simulink model "ASM_Traffic_A11"  (R2026a)
settings: Solver=ode1  StartTime=SIM.tstart.v  StopTime=SIM.tend.v  FixedStep=SIM.StepSize.v
PostLoadFcn:
  | if any(exist('dsrtsu_mdlpostloadfcn', 'file') ~= 0), dsrtsu_mdlpostloadfcn('Execute', bdroot); end
  | try, asm_mdl_postloadfcn(bdroot, 'UpdateModel', 3600); catch, disp(lasterr); end,
InitFcn:
  | , if any(exist('rtifpga_mdlclblib', 'file') ~= 0), rtifpga_mdlclblib('Init', bdroot); end,
  | , if any(exist('dsmpb_private', 'file') ~= 0), dsmpb_private('dsmpb_mdlclblib', 'Init', bdroot); end,
undefined symbols (not defined in the file): _to_, a0b2, ASM_BrakeHydraulics_DemoSystems, ASM_VehicleDynamics_DemoSystems, b98103fe8ad365046cd0, BrakeCircuit, controllerConfig, CPT, Crankshaft, DiscIntNeverNeededParam, dsmsi, FinalDriveAssembly, instance, MDL, ModeSignals, mu, Pos_BrakePedal_Maneuver, rad, RefSignals, s_to_rpm, SIM, SoftECU, Suspension, Tire, Transmission
libraries: ASM_Traffic_lib x135, simulink x98, ASM_Utils_lib x77, ASM_VehicleDynamics_lib x70, ASM_Environment_lib x22, dsmpblib x20, dsmsilib x15, MDLD_Utils_lib x10, ASM_BrakeHydraulics_lib x3, sl_discontinuities x2
(part 34 of 63)

== system ASM_Traffic_A11/DomainControl/DriverAssistance/Interface_In/ModelSignals/m_TotalVehicle[kg]_ ==
  In1 : Inport
  Gain : Gain  SaturateOnIntegerOverflow=on  OutDataTypeStr=Inherit: Same as input  ParamDataTypeStr=Inherit: Same as input
  Out1 : Outport  VectorParamsAs1DForOutWhenUnconnected=off
  wires:
  In1/1 -> Gain/1
  Gain/1 -> Out1/1

== system ASM_Traffic_A11/DomainControl/DriverAssistance/Interface_In/ModelSignals/r_Dyn_Tire[FL;FR;RL;RR][m]_ ==
  In1 : Inport
  Gain : Gain  SaturateOnIntegerOverflow=on  OutDataTypeStr=Inherit: Same as input  ParamDataTypeStr=Inherit: Same as input
  Out1 : Outport  VectorParamsAs1DForOutWhenUnconnected=off
  wires:
  In1/1 -> Gain/1
  Gain/1 -> Out1/1

== system ASM_Traffic_A11/DomainControl/DriverAssistance/Interface_In/ModelSignals/s_Fellows_Ref[m]_ ==
  In1 : Inport
  Gain : Gain  SaturateOnIntegerOverflow=on  OutDataTypeStr=Inherit: Same as input  ParamDataTypeStr=Inherit: Same as input
  Out1 : Outport  VectorParamsAs1DForOutWhenUnconnected=off
  wires:
  In1/1 -> Gain/1
  Gain/1 -> Out1/1

== system ASM_Traffic_A11/DomainControl/DriverAssistance/Interface_In/ModelSignals/s_Vehicle_Road[m]_ ==
  In1 : Inport
  Gain : Gain  SaturateOnIntegerOverflow=on  OutDataTypeStr=Inherit: Same as input  ParamDataTypeStr=Inherit: Same as input
  Out1 : Outport  VectorParamsAs1DForOutWhenUnconnected=off
  wires:
  In1/1 -> Gain/1
  Gain/1 -> Out1/1

== system ASM_Traffic_A11/DomainControl/DriverAssistance/Interface_In/ModelSignals/v_Rel_Fellows[m|s]_ ==
  In1 : Inport
  Gain : Gain  SaturateOnIntegerOverflow=on  OutDataTypeStr=Inherit: Same as input  ParamDataTypeStr=Inherit: Same as input
  Out1 : Outport  VectorParamsAs1DForOutWhenUnconnected=off
  wires:
  In1/1 -> Gain/1
  Gain/1 -> Out1/1

== system ASM_Traffic_A11/DomainControl/DriverAssistance/Interface_In/ModelSignals/v_Vehicle[km|h]_ ==
  In1 : Inport
  Gain : Gain  SaturateOnIntegerOverflow=on  OutDataTypeStr=Inherit: Same as input  ParamDataTypeStr=Inherit: Same as input
  Out1 : Outport  VectorParamsAs1DForOutWhenUnconnected=off
  wires:
  In1/1 -> Gain/1
  Gain/1 -> Out1/1

== system ASM_Traffic_A11/DomainControl/DriverAssistance/Interface_In/ModelSignals/v_x_Vehicle_CoG[km|h]_ ==
  In1 : Inport
  Gain : Gain  SaturateOnIntegerOverflow=on  OutDataTypeStr=Inherit: Same as input  ParamDataTypeStr=Inherit: Same as input
  Out1 : Outport  VectorParamsAs1DForOutWhenUnconnected=off
  wires:
  In1/1 -> Gain/1
  Gain/1 -> Out1/1

== system ASM_Traffic_A11/DomainControl/DriverAssistance/Interface_Out/Animation/Dist_Long[m]_ ==
  In1 : Inport
  Gain : Gain  SaturateOnIntegerOverflow=on  OutDataTypeStr=Inherit: Same as input  ParamDataTypeStr=Inherit: Same as input
  Out1 : Outport  VectorParamsAs1DForOutWhenUnconnected=off
  wires:
  In1/1 -> Gain/1
  Gain/1 -> Out1/1

== system ASM_Traffic_A11/DomainControl/DriverAssistance/Interface_Out/Animation/Distance_Set[m]_ ==
  In1 : Inport
  Gain : Gain  SaturateOnIntegerOverflow=on  OutDataTypeStr=Inherit: Same as input  ParamDataTypeStr=Inherit: Same as input
  Out1 : Outport  VectorParamsAs1DForOutWhenUnconnected=off
  wires:
  In1/1 -> Gain/1
  Gain/1 -> Out1/1

== system ASM_Traffic_A11/DomainControl/DriverAssistance/Interface_Out/Animation/State_ACC[0Off|1On]_ ==
  In1 : Inport
  Gain : Gain  SaturateOnIntegerOverflow=on  OutDataTypeStr=Inherit: Same as input  ParamDataTypeStr=Inherit: Same as input
  Out1 : Outport  VectorParamsAs1DForOutWhenUnconnected=off
  wires:
  In1/1 -> Gain/1
  Gain/1 -> Out1/1

== system ASM_Traffic_A11/DomainControl/DriverAssistance/Interface_Out/Animation/Target_Detected[0|1]_ ==
  In1 : Inport
  Gain : Gain  SaturateOnIntegerOverflow=on  OutDataTypeStr=Inherit: Same as input  ParamDataTypeStr=Inherit: Same as input
  Out1 : Outport  VectorParamsAs1DForOutWhenUnconnected=off
  wires:
  In1/1 -> Gain/1
  Gain/1 -> Out1/1

== system ASM_Traffic_A11/DomainControl/DriverAssistance/Interface_Out/Animation/v_Set[km|h]_ ==
  In1 : Inport
  Gain : Gain  SaturateOnIntegerOverflow=on  OutDataTypeStr=Inherit: Same as input  ParamDataTypeStr=Inherit: Same as input
  Out1 : Outport  VectorParamsAs1DForOutWhenUnconnected=off
  wires:
  In1/1 -> Gain/1
  Gain/1 -> Out1/1

== system ASM_Traffic_A11/DomainControl/DriverAssistance/Interface_Out/Control_ModelSignals/ACC_State[1OFF|2Standby|3ON]_ ==
  In1 : Inport
  Gain : Gain  SaturateOnIntegerOverflow=on  OutDataTypeStr=Inherit: Same as input  ParamDataTypeStr=Inherit: Same as input
  Out1 : Outport  VectorParamsAs1DForOutWhenUnconnected=off
  wires:
  Gain/1 -> Out1/1
  In1/1 -> Gain/1

== system ASM_Traffic_A11/DomainControl/DriverAssistance/Interface_Out/Control_ModelSignals/AEB[0|1]_ ==
  In1 : Inport
  Gain : Gain  SaturateOnIntegerOverflow=on  OutDataTypeStr=Inherit: Same as input  ParamDataTypeStr=Inherit: Same as input
  Out1 : Outport  VectorParamsAs1DForOutWhenUnconnected=off
  wires:
  In1/1 -> Gain/1
  Gain/1 -> Out1/1

== system ASM_Traffic_A11/DomainControl/DriverAssistance/Interface_Out/Control_ModelSignals/Driver_Override_ACC_Active[0Off|1On]_ ==
  In1 : Inport
  Gain : Gain  SaturateOnIntegerOverflow=on  OutDataTypeStr=Inherit: Same as input  ParamDataTypeStr=Inherit: Same as input
  Out1 : Outport  VectorParamsAs1DForOutWhenUnconnected=off
  wires:
  Gain/1 -> Out1/1
  In1/1 -> Gain/1

== system ASM_Traffic_A11/DomainControl/DriverAssistance/Interface_Out/Control_ModelSignals/Driver_Override_ACC_Reason[0NoOverride|1BrakePedal|2AccPedal]_ ==
  In1 : Inport
  Gain : Gain  SaturateOnIntegerOverflow=on  OutDataTypeStr=Inherit: Same as input  ParamDataTypeStr=Inherit: Same as input
  Out1 : Outport  VectorParamsAs1DForOutWhenUnconnected=off
  wires:
  Gain/1 -> Out1/1
  In1/1 -> Gain/1

== system ASM_Traffic_A11/DomainControl/DriverAssistance/Interface_Out/Control_ModelSignals/Enable_Trq_Decrease_ACC[0|1]_ ==
  In1 : Inport
  Gain : Gain  SaturateOnIntegerOverflow=on  OutDataTypeStr=Inherit: Same as input  ParamDataTypeStr=Inherit: Same as input
  Out1 : Outport  VectorParamsAs1DForOutWhenUnconnected=off
  wires:
  In1/1 -> Gain/1
  Gain/1 -> Out1/1

== system ASM_Traffic_A11/DomainControl/DriverAssistance/Interface_Out/Control_ModelSignals/Enable_Trq_Increase_ACC[0|1]_ ==
  In1 : Inport
  Gain : Gain  SaturateOnIntegerOverflow=on  OutDataTypeStr=Inherit: Same as input  ParamDataTypeStr=Inherit: Same as input
  Out1 : Outport  VectorParamsAs1DForOutWhenUnconnected=off
  wires:
  In1/1 -> Gain/1
  Gain/1 -> Out1/1

== system ASM_Traffic_A11/DomainControl/DriverAssistance/Interface_Out/Control_ModelSignals/FCW[0|1]_ ==
  In1 : Inport
  Gain : Gain  SaturateOnIntegerOverflow=on  OutDataTypeStr=Inherit: Same as input  ParamDataTypeStr=Inherit: Same as input
  Out1 : Outport  VectorParamsAs1DForOutWhenUnconnected=off
  wires:
  In1/1 -> Gain/1
  Gain/1 -> Out1/1

== system ASM_Traffic_A11/DomainControl/DriverAssistance/Interface_Out/Control_ModelSignals/Trq_DecreaseRequest_ACC[Nm]_ ==
  In1 : Inport
  Gain : Gain  SaturateOnIntegerOverflow=on  OutDataTypeStr=Inherit: Same as input  ParamDataTypeStr=Inherit: Same as input
  Out1 : Outport  VectorParamsAs1DForOutWhenUnconnected=off
  wires:
  In1/1 -> Gain/1
  Gain/1 -> Out1/1

== system ASM_Traffic_A11/DomainControl/DriverAssistance/Interface_Out/Control_ModelSignals/Trq_IncreaseRequest_ACC[Front;Rear][Nm]_ ==
  In1 : Inport
  Gain : Gain  SaturateOnIntegerOverflow=on  OutDataTypeStr=Inherit: Same as input  ParamDataTypeStr=Inherit: Same as input
  Out1 : Outport  VectorParamsAs1DForOutWhenUnconnected=off
  wires:
  In1/1 -> Gain/1
  Gain/1 -> Out1/1

== system ASM_Traffic_A11/DomainControl/DriverAssistance/Interface_Out/Control_ModelSignals/Trq_IncreaseRequest_ACC[Nm]_ ==
  In1 : Inport
  Gain : Gain  SaturateOnIntegerOverflow=on  OutDataTypeStr=Inherit: Same as input  ParamDataTypeStr=Inherit: Same as input
  Out1 : Outport  VectorParamsAs1DForOutWhenUnconnected=off
  wires:
  In1/1 -> Gain/1
  Gain/1 -> Out1/1

== system ASM_Traffic_A11/DomainControl/DriverAssistance/SignalInterface/ASMSignalInterface/signal_structure ==
  ASMSignalBus : Inport
  BusSelector_1 : BusSelector  OutputSignals=Controller_ACC,Interface_ACC,Operator_Interface_ACC,Target_Selection_ACC
  ContentID : Constant  Value=814723687
  Controller_ACC : BusSelector  OutputSignals=State_ACC[0Off|1On],Sw_ACC_Distance[s],Control_Mode_ACC[0Off|1CC|2DC],v_Set_CC[km|h],v_Set_DC[km|h],v_Set[km|h],a_x_Set[m|s2],a_x_UpperLimit[m|s2],a_x_LowerLimit[m|s2],a_x_RisingRateMax[m|s3],a_x_FallingRateMax[m|s3]s,Distance_Set[m],Dist_Ref_Vehicle[m],FCW[0Off|1On],AEB[0Off|1On],TTC[s],Collision[0Off|1On],Sw_BrakeMode[1Comfort|2AEBOnly|3AEBOff],Enable_Trq_Brake_ACC[0|1],Enable_Trq_Engine_ACC[0|1]
  DataTypeConversion_17 : DataTypeConversion  OutDataTypeStr=double
  InfoBlock : Subsystem
      mask Display: fprintf('Structural changes of the signal bus require an update \nof the ''ASMSignalCollector'' block. \n\nTo start the update process double click the parent block.\n\n WARNING:\n During update this subsystem will be cleared completely')
  Interface_ACC : BusSelector  OutputSignals=Trq_Request_Engine_ACC[Nm],Trq_Request_Engine_ACC[Front;Rear][Nm],Trq_Request_Brake_ACC[Nm]
  MDLD_DATA_CAPTURE : MDLD_Utils_lib/ModelDeskPlotInterface/DataCapture_Sfcn/MDLD_DATA_CAPTURE  inputPortWidth=70  measurementSignals=[0 0 0 0 0 0 0 0 0 0 0 0 0 0 0 0 0 0 0 0 0 0 0 0 0 0 0 0 0 0 0 0 0 0 0 0 0 0 0 0 0 0 0 0 0 0 0 0 0 0 0 0 0 0 0 0 0 0 0 0 0 0 0 0 0 0 0 0 0 0]  downsampling=1  samplingPeriod=SIM.StepSize.v  uuid=0  ASMProperties=struct('Name','mdld_data_capture','Version','1.0','Library','mdld_utils_lib')  startTriggerDelay=0  startTriggerLogic=0  startTriggerCount=0  startTriggerConditions=[0,0,0,0,0,0,0,0,0]  stopTriggerDelay=0  stopTriggerLogic=0  stopTriggerCount=0  stopTriggerConditions=[0,0,0,0,0,0,0,0,0]  ContentID_RefStruct=814723687
  Operator_Interface_ACC : BusSelector  OutputSignals=Sw_ACC_On[0Off|1On],Sw_ACC_Off[0Off|1On],Sw_ACC_Cancel[0Off|1On],Sw_ACC_Resume[0Off|1On],Sw_ACC_Speed_Set[0Off|1On],Sw_ACC_Speed_Increase[0Off|1On],Sw_ACC_Speed_Decrease[0Off|1On],ACC_State[1OFF|2Standby|3ON],Driver_Override_ACC_Active[0Off|1On],Driver_Override_ACC_Reason[0NoOverride|1BrakePedal|2AccPedal],V_Set_CruiseControl[km|h]
  Reshape_22 : Reshape
  Reshape_38 : Reshape
  Reshape_39 : Reshape
  SignalFilter : Mux  Inputs=41
  SignalFilterGain : Gain
  Target_Selection_ACC : BusSelector  OutputSignals=Target_Detected[0|1],Dist_Long[m],v_Rel[m|s],InLaneCheck[0|1],LaneCrossingCheck[0|1],v_Rel_Road[m|s],s_Fellows_Near[m]
  Terminator : Terminator
  wires:
  ASMSignalBus/1 -> BusSelector_1/1
  BusSelector_1/1 -> Controller_ACC/1  "<Controller_ACC>"
  BusSelector_1/2 -> Interface_ACC/1  "<Interface_ACC>"
  BusSelector_1/3 -> Operator_Interface_ACC/1  "<Operator_Interface_ACC>"
  BusSelector_1/4 -> Target_Selection_ACC/1  "<Target_Selection_ACC>"
  ContentID/1 -> Terminator/1
  Controller_ACC/1 -> SignalFilter/1  "<State_ACC[0Off|1On]>"
  Controller_ACC/2 -> SignalFilter/2  "<Sw_ACC_Distance[s]>"
  Controller_ACC/3 -> SignalFilter/3  "<Control_Mode_ACC[0Off|1CC|2DC]>"
  Controller_ACC/4 -> SignalFilter/4  "<v_Set_CC[km|h]>"
  Controller_ACC/5 -> SignalFilter/5  "<v_Set_DC[km|h]>"
  Controller_ACC/6 -> SignalFilter/6  "<v_Set[km|h]>"
  Controller_ACC/7 -> SignalFilter/7  "<a_x_Set[m|s2]>"
  Controller_ACC/8 -> SignalFilter/8  "<a_x_UpperLimit[m|s2]>"
  Controller_ACC/9 -> SignalFilter/9  "<a_x_LowerLimit[m|s2]>"
  Controller_ACC/10 -> SignalFilter/10  "<a_x_RisingRateMax[m|s3]>"
  Controller_ACC/11 -> SignalFilter/11  "<a_x_FallingRateMax[m|s3]s>"
  Controller_ACC/12 -> SignalFilter/12  "<Distance_Set[m]>"
  Controller_ACC/13 -> SignalFilter/13  "<Dist_Ref_Vehicle[m]>"
  Controller_ACC/14 -> SignalFilter/14  "<FCW[0Off|1On]>"
  Controller_ACC/15 -> SignalFilter/15  "<AEB[0Off|1On]>"
  Controller_ACC/16 -> SignalFilter/16  "<TTC[s]>"
  Controller_ACC/17 -> DataTypeConversion_17/1  "<Collision[0Off|1On]>"
  DataTypeConversion_17/1 -> SignalFilter/17
  Controller_ACC/18 -> SignalFilter/18  "<Sw_BrakeMode[1Comfort|2AEBOnly|3AEBOff]>"
  Controller_ACC/19 -> SignalFilter/19  "<Enable_Trq_Brake_ACC[0|1]>"
  Controller_ACC/20 -> SignalFilter/20  "<Enable_Trq_Engine_ACC[0|1]>"
  Interface_ACC/1 -> SignalFilter/21  "<Trq_Request_Engine_ACC[Nm]>"
  Interface_ACC/2 -> Reshape_22/1  "<Trq_Request_Engine_ACC[Front;Rear][Nm]>"
  Reshape_22/1 -> SignalFilter/22
  Interface_ACC/3 -> SignalFilter/23  "<Trq_Request_Brake_ACC[Nm]>"
  Operator_Interface_ACC/1 -> SignalFilter/24  "<Sw_ACC_On[0Off|1On]>"
  Operator_Interface_ACC/2 -> SignalFilter/25  "<Sw_ACC_Off[0Off|1On]>"
  Operator_Interface_ACC/3 -> SignalFilter/26  "<Sw_ACC_Cancel[0Off|1On]>"
  Operator_Interface_ACC/4 -> SignalFilter/27  "<Sw_ACC_Resume[0Off|1On]>"
  Operator_Interface_ACC/5 -> SignalFilter/28  "<Sw_ACC_Speed_Set[0Off|1On]>"
  Operator_Interface_ACC/6 -> SignalFilter/29  "<Sw_ACC_Speed_Increase[0Off|1On]>"
  Operator_Interface_ACC/7 -> SignalFilter/30  "<Sw_ACC_Speed_Decrease[0Off|1On]>"
  Operator_Interface_ACC/8 -> SignalFilter/31  "<ACC_State[1OFF|2Standby|3ON]>"
  Operator_Interface_ACC/9 -> SignalFilter/32  "<Driver_Override_ACC_Active[0Off|1On]>"
  Operator_Interface_ACC/10 -> SignalFilter/33  "<Driver_Override_ACC_Reason[0NoOverride|1BrakePedal|2AccPedal]>"
  Operator_Interface_ACC/11 -> SignalFilter/34  "<V_Set_CruiseControl[km|h]>"
  Target_Selection_ACC/1 -> SignalFilter/35  "<Target_Detected[0|1]>"
  Target_Selection_ACC/2 -> SignalFilter/36  "<Dist_Long[m]>"
  Target_Selection_ACC/3 -> SignalFilter/37  "<v_Rel[m|s]>"
  Target_Selection_ACC/4 -> Reshape_38/1  "<InLaneCheck[0|1]>"
  Reshape_38/1 -> SignalFilter/38
  Target_Selection_ACC/5 -> Reshape_39/1  "<LaneCrossingCheck[0|1]>"
  Reshape_39/1 -> SignalFilter/39
  Target_Selection_ACC/6 -> SignalFilter/40  "<v_Rel_Road[m|s]>"
  Target_Selection_ACC/7 -> SignalFilter/41  "<s_Fellows_Near[m]>"
  SignalFilter/1 -> SignalFilterGain/1
  SignalFilterGain/1 -> MDLD_DATA_CAPTURE/1

== system ASM_Traffic_A11/DomainControl/DriverAssistance/SignalInterface/ExternalOutports/Select_Outport_Signals ==
  ASMSignalBus : Inport
  Bus Selector : BusSelector  OutputSignals=Controller_ACC,Interface_ACC,Operator_Interface_ACC,Target_Selection_ACC
  Controller_ACC : Outport  VectorParamsAs1DForOutWhenUnconnected=off
  Interface_ACC : Outport  Port=2  VectorParamsAs1DForOutWhenUnconnected=off
  Operator_Interface_ACC : Outport  Port=3  VectorParamsAs1DForOutWhenUnconnected=off
  Target_Selection_ACC : Outport  Port=4  VectorParamsAs1DForOutWhenUnconnected=off
  wires:
  ASMSignalBus/1 -> Bus Selector/1
  Bus Selector/1 -> Controller_ACC/1  "<Controller_ACC>"
  Bus Selector/2 -> Interface_ACC/1  "<Interface_ACC>"
  Bus Selector/3 -> Operator_Interface_ACC/1  "<Operator_Interface_ACC>"
  Bus Selector/4 -> Target_Selection_ACC/1  "<Target_Selection_ACC>"

== system ASM_Traffic_A11/DomainControl/StartSystem/Control/SoftECU_StartSystem/ASMSignalCollector ==
  Bus Creator1 : BusCreator  Inputs=1
  ASMSIgnalBus : Outport  VectorParamsAs1DForOutWhenUnconnected=off
  wires:
  [ASMBUS_START_BUTTON] -> Bus Creator1/1
  Bus Creator1/1 -> ASMSIgnalBus/1  "Control"

== system ASM_Traffic_A11/DomainControl/StartSystem/Control/SoftECU_StartSystem/DisableReset ==
  note: Start button is not reset, if crankshaft reset is disabled
  Reset_VehicleStates[0|1] : Inport
  Sw_CrankShaft_Reset[0Disabled|1Enabled] : Inport  Port=2
  MultiPortSwitch : MultiPortSwitch  DataPortOrder=Zero-based contiguous  Inputs=2  zeroidx=on
  NO_Reset : Constant  Value=0
  Reset[0|1] : Outport  VectorParamsAs1DForOutWhenUnconnected=off
  wires:
  MultiPortSwitch/1 -> Reset[0|1]/1
  Sw_CrankShaft_Reset[0Disabled|1Enabled]/1 -> MultiPortSwitch/1
  NO_Reset/1 -> MultiPortSwitch/2
  Reset_VehicleStates[0|1]/1 -> MultiPortSwitch/3

== system ASM_Traffic_A11/DomainControl/StartSystem/Control/Sw_ECU_Signals/State_StartButton[-2|-1|0|1|2|3] ==
  SoftECU : Inport
  RealECU : Inport  Port=2
  Const_State_StartButton[-2|-1|0|1|2|3] : Constant  Value=0
  MultiPortSwitch : MultiPortSwitch
  Sw_State_StartButton[1SoftECU|2RealECU|3Const] : Constant  Value=CPT.MDL_SW.Sw_State_StartButton.v
  State_StartButton[-2|-1|0|1|2|3] : Outport  VectorParamsAs1DForOutWhenUnconnected=off
  wires:
  Sw_State_StartButton[1SoftECU|2RealECU|3Const]/1 -> MultiPortSwitch/1
  SoftECU/1 -> MultiPortSwitch/2
  RealECU/1 -> MultiPortSwitch/3
  Const_State_StartButton[-2|-1|0|1|2|3]/1 -> MultiPortSwitch/4
  MultiPortSwitch/1 -> State_StartButton[-2|-1|0|1|2|3]/1

== system ASM_Traffic_A11/DomainControl/StartSystem/Control/Sw_ECU_Signals/Sw_Ignition[0|1] ==
  SoftECU : Inport
  RealECU : Inport  Port=2
  Const_Sw_Ignition[0|1] : Constant  Value=0
  MultiPortSwitch : MultiPortSwitch
  Sw_Ignition[1SoftECU|2RealECU|3Const] : Constant  Value=CPT.MDL_SW.Sw_Ignition.v
  Sw_Ignition[0|1] : Outport  VectorParamsAs1DForOutWhenUnconnected=off
  wires:
  MultiPortSwitch/1 -> Sw_Ignition[0|1]/1
  Const_Sw_Ignition[0|1]/1 -> MultiPortSwitch/4
  RealECU/1 -> MultiPortSwitch/3
  SoftECU/1 -> MultiPortSwitch/2
  Sw_Ignition[1SoftECU|2RealECU|3Const]/1 -> MultiPortSwitch/1

== system ASM_Traffic_A11/DomainControl/StartSystem/Control/Sw_ECU_Signals/Sw_StarterReq[0|1] ==
  SoftECU : Inport
  RealECU : Inport  Port=2
  Const_Sw_StarterReq[0|1] : Constant  Value=0
  MultiPortSwitch : MultiPortSwitch
  Sw_StarterReq[1SoftECU|2RealECU|3Const] : Constant  Value=CPT.MDL_SW.Sw_StarterReq.v
  Sw_StarterReq[0|1] : Outport  VectorParamsAs1DForOutWhenUnconnected=off
  wires:
  Sw_StarterReq[1SoftECU|2RealECU|3Const]/1 -> MultiPortSwitch/1
  SoftECU/1 -> MultiPortSwitch/2
  RealECU/1 -> MultiPortSwitch/3
  Const_Sw_StarterReq[0|1]/1 -> MultiPortSwitch/4
  MultiPortSwitch/1 -> Sw_StarterReq[0|1]/1

== system ASM_Traffic_A11/DomainControl/StartSystem/Control/UserInterface/ASMSignalBus_Control ==
  In : Inport
  Terminator_1 : Terminator
  tag scope: ASMBUS_StartSystem_Control=global
  wires:
  In/1 -> [ASMBUS_StartSystem_Control]  "Control"
  [ASMBUS_StartSystem_Control] -> Terminator_1/1

== system ASM_Traffic_A11/DomainControl/StartSystem/Control/UserInterface/DISP_Control ==
  In : Inport
  Interface_In : Inport  Port=2
  Bus Selector1 : BusSelector  OutputSignals=ExternalModel.State_Engine[0|1|2|3|4],ExternalModel.Mode_StartButtonState[1Stim|2SoftECU]
  Bus Selector3 : BusSelector  OutputSignals=StartButton.Flag_NotPressed_Pedal[0|1],StartButton.Sw_Ignition[0|1],StartButton.Sw_StarterReq[0|1],StartButton.State_StartButton[-2|-1|0|1|2|3]
  Flag_NotPressed_Pedal[0|1] : Subsystem
      mask Display: disp('')
  START_BUTTON : Scope  NumInputPorts=4
      settings: TimeSpan=5  DataLoggingMaxPoints=20000  DataLoggingDecimation=10  DataLoggingSaveFormat=Array
  StartStateButtonLogic : Subsystem
  State_StartButton[-2NotAuthorized|-1PowerOff|0Acc|1PowerOn|2StarterOn|3EngRunning] : Subsystem
      mask Display: disp('')
  Sw_Ignition[0|1] : Subsystem
      mask Display: disp('')
  Sw_StarterReq[0|1] : Subsystem
      mask Display: disp('')
  wires:
  Bus Selector3/3 -> Sw_StarterReq[0|1]/1(In1)  "<Sw_StarterReq[0|1]>"
  Bus Selector1/1 -> StartStateButtonLogic/2(State_Engine[0|1|2|3|4])  "<State_Engine[0|1|2|3|4]>"
  Bus Selector1/2 -> StartStateButtonLogic/3(Mode_StartButtonState[1Stim|2SoftECU])  "<Mode_StartButtonState[1Stim|2SoftECU]>"
  Flag_NotPressed_Pedal[0|1]/1(Out1) -> START_BUTTON/1  "Flag_NotPressed_Pedal[0|1]"
  StartStateButtonLogic/1(Out1) -> State_StartButton[-2NotAuthorized|-1PowerOff|0Acc|1PowerOn|2StarterOn|3EngRunning]/1(In1)
  State_StartButton[-2NotAuthorized|-1PowerOff|0Acc|1PowerOn|2StarterOn|3EngRunning]/1(Out1) -> START_BUTTON/4  "State_StartButton[-2NotAuthorized|-1PowerOff|0Acc|1PowerOn|2StarterOn|3EngRunning]"
  Sw_Ignition[0|1]/1(Out1) -> START_BUTTON/2  "Sw_Ignition[0|1]"
  Bus Selector3/2 -> Sw_Ignition[0|1]/1(In1)  "<Sw_Ignition[0|1]>"
  Sw_StarterReq[0|1]/1(Out1) -> START_BUTTON/3  "Sw_StarterReq[0|1]"
  Bus Selector3/4 -> StartStateButtonLogic/1(State_StartButton[-2|-1|0|1|2|3])  "<State_StartButton[-2|-1|0|1|2|3]>"
  Bus Selector3/1 -> Flag_NotPressed_Pedal[0|1]/1(In1)  "<Flag_NotPressed_Pedal[0|1]>"
  In/1 -> Bus Selector3/1
  Interface_In/1 -> Bus Selector1/1

== system ASM_Traffic_A11/DomainControl/StartSystem/Control/UserInterface/PAR_Control ==
  Bus Creator2 : BusCreator  Inputs=1
  State_KeyFob[1NotAuthorized|2Authorized] : Constant  Value=2
  Out : Outport  VectorParamsAs1DForOutWhenUnconnected=off
  wires:
  Bus Creator2/1 -> Out/1  "PAR2Control"
  State_KeyFob[1NotAuthorized|2Authorized]/1 -> Bus Creator2/1  "State_KeyFob[1NotAuthorized|2Authorized]"

== system ASM_Traffic_A11/DomainControl/StartSystem/Interface_In/ExternalSignals/ExternalECU_StartSystem ==
  State_StartButton[-2|-1|0|1|2|3] : Inport
  Sw_Ignition[0|1] : Inport  Port=2
  Sw_StarterReq[0|1] : Inport  Port=3
  Bus Creator4 : BusCreator  Inputs=3
  Out : Outport  VectorParamsAs1DForOutWhenUnconnected=off
  wires:
  State_StartButton[-2|-1|0|1|2|3]/1 -> Bus Creator4/1  "State_StartButton[-2|-1|0|1|2|3]"
  Bus Creator4/1 -> Out/1  "ExternalECU"
  Sw_Ignition[0|1]/1 -> Bus Creator4/2  "Sw_Ignition[0|1]"
  Sw_StarterReq[0|1]/1 -> Bus Creator4/3  "Sw_StarterReq[0|1]"

== system ASM_Traffic_A11/DomainControl/StartSystem/Interface_In/ModelSignals/Mode_StartButtonState[1Stim|2SoftECU]_ ==
  In1 : Inport
  DummyGain : Gain  SaturateOnIntegerOverflow=on  OutDataTypeStr=Inherit: Same as input  ParamDataTypeStr=Inherit: Same as input
  Out1 : Outport  VectorParamsAs1DForOutWhenUnconnected=off
  wires:
  In1/1 -> DummyGain/1
  DummyGain/1 -> Out1/1

== system ASM_Traffic_A11/DomainControl/StartSystem/Interface_In/ModelSignals/Mode_Transmission[1Manual|2Automatic]_ ==
  In1 : Inport
  DummyGain : Gain  SaturateOnIntegerOverflow=on  OutDataTypeStr=Inherit: Same as input  ParamDataTypeStr=Inherit: Same as input
  Out1 : Outport  VectorParamsAs1DForOutWhenUnconnected=off
  wires:
  In1/1 -> DummyGain/1
  DummyGain/1 -> Out1/1

== system ASM_Traffic_A11/DomainControl/StartSystem/Interface_In/ModelSignals/Pos_BrakePedal[%]_ ==
  In1 : Inport
  DummyGain : Gain  SaturateOnIntegerOverflow=on  OutDataTypeStr=Inherit: Same as input  ParamDataTypeStr=Inherit: Same as input
  Out1 : Outport  VectorParamsAs1DForOutWhenUnconnected=off
  wires:
  In1/1 -> DummyGain/1
  DummyGain/1 -> Out1/1

== system ASM_Traffic_A11/DomainControl/StartSystem/Interface_In/ModelSignals/Pos_ClutchPedal[%]_ ==
  In1 : Inport
  DummyGain : Gain  SaturateOnIntegerOverflow=on  OutDataTypeStr=Inherit: Same as input  ParamDataTypeStr=Inherit: Same as input
  Out1 : Outport  VectorParamsAs1DForOutWhenUnconnected=off
  wires:
  In1/1 -> DummyGain/1
  DummyGain/1 -> Out1/1

== system ASM_Traffic_A11/DomainControl/StartSystem/Interface_In/ModelSignals/Reset_States[0|1]_ ==
  In1 : Inport
  DummyGain : Gain  SaturateOnIntegerOverflow=on  OutDataTypeStr=Inherit: Same as input  ParamDataTypeStr=Inherit: Same as input
  Out1 : Outport  VectorParamsAs1DForOutWhenUnconnected=off
  wires:
  In1/1 -> DummyGain/1
  DummyGain/1 -> Out1/1

== system ASM_Traffic_A11/DomainControl/StartSystem/Interface_In/ModelSignals/SelectorLever[-3T|-2P|-1R|0N|1D]_ ==
  In1 : Inport
  DummyGain : Gain  SaturateOnIntegerOverflow=on  OutDataTypeStr=Inherit: Same as input  ParamDataTypeStr=Inherit: Same as input
  Out1 : Outport  VectorParamsAs1DForOutWhenUnconnected=off
  wires:
  In1/1 -> DummyGain/1
  DummyGain/1 -> Out1/1

== system ASM_Traffic_A11/DomainControl/StartSystem/Interface_In/ModelSignals/State_Engine[0|1|2|3|4]_ ==
  In1 : Inport
  DummyGain : Gain  SaturateOnIntegerOverflow=on  OutDataTypeStr=Inherit: Same as input  ParamDataTypeStr=Inherit: Same as input
  Out1 : Outport  VectorParamsAs1DForOutWhenUnconnected=off
  wires:
  In1/1 -> DummyGain/1
  DummyGain/1 -> Out1/1

== system ASM_Traffic_A11/DomainControl/StartSystem/Interface_In/ModelSignals/State_StartButton[-1PowerOff|0Acc|1PowerOn|2StarterOn]_ ==
  In1 : Inport
  DummyGain : Gain  SaturateOnIntegerOverflow=on  OutDataTypeStr=Inherit: Same as input  ParamDataTypeStr=Inherit: Same as input
  Out1 : Outport  VectorParamsAs1DForOutWhenUnconnected=off
  wires:
  In1/1 -> DummyGain/1
  DummyGain/1 -> Out1/1

== system ASM_Traffic_A11/DomainControl/StartSystem/Interface_In/ModelSignals/Sw_CrankShaft_Reset[0Disabled|1Enabled]_ ==
  In1 : Inport
  DummyGain : Gain  SaturateOnIntegerOverflow=on  OutDataTypeStr=Inherit: Same as input  ParamDataTypeStr=Inherit: Same as input
  Out1 : Outport  VectorParamsAs1DForOutWhenUnconnected=off
  wires:
  DummyGain/1 -> Out1/1
  In1/1 -> DummyGain/1

== system ASM_Traffic_A11/DomainControl/StartSystem/Interface_In/ModelSignals/Sw_ModelDeskPlottingInterface[0Disabled|1Enabled]_ ==
  In1 : Inport
  Gain : Gain
  Out1 : Outport
  wires:
  Gain/1 -> Out1/1
  In1/1 -> Gain/1

== system ASM_Traffic_A11/DomainControl/StartSystem/Interface_In/ModelSignals/Sw_ModelPortBlocks[0Disabled|1Enabled]_ ==
  In1 : Inport
  Gain : Gain
  Out1 : Outport
  wires:
  Gain/1 -> Out1/1
  In1/1 -> Gain/1

== system ASM_Traffic_A11/DomainControl/StartSystem/Interface_In/ModelSignals/Sw_StartButton[0Off|1On]_ ==
  In1 : Inport
  DummyGain : Gain  SaturateOnIntegerOverflow=on  OutDataTypeStr=Inherit: Same as input  ParamDataTypeStr=Inherit: Same as input
  Out1 : Outport  VectorParamsAs1DForOutWhenUnconnected=off
  wires:
  In1/1 -> DummyGain/1
  DummyGain/1 -> Out1/1

== system ASM_Traffic_A11/DomainControl/StartSystem/Interface_Out/Control_ModelSignals/State_StartButton[-2|-1|0|1|2|3]_ ==
  In1 : Inport
  DummyGain : Gain  SaturateOnIntegerOverflow=on  OutDataTypeStr=Inherit: Same as input  ParamDataTypeStr=Inherit: Same as input
  Out1 : Outport  VectorParamsAs1DForOutWhenUnconnected=off
  wires:
  DummyGain/1 -> Out1/1
  In1/1 -> DummyGain/1

== system ASM_Traffic_A11/DomainControl/StartSystem/Interface_Out/Control_ModelSignals/Sw_Ignition[0|1]_ ==
  In1 : Inport
  DummyGain : Gain  SaturateOnIntegerOverflow=on  OutDataTypeStr=Inherit: Same as input  ParamDataTypeStr=Inherit: Same as input
  Out1 : Outport  VectorParamsAs1DForOutWhenUnconnected=off
  wires:
  DummyGain/1 -> Out1/1
  In1/1 -> DummyGain/1

== system ASM_Traffic_A11/DomainControl/StartSystem/Interface_Out/Control_ModelSignals/Sw_StarterReq[0|1]_ ==
  In1 : Inport
  DummyGain : Gain  SaturateOnIntegerOverflow=on  OutDataTypeStr=Inherit: Same as input  ParamDataTypeStr=Inherit: Same as input
  Out1 : Outport  VectorParamsAs1DForOutWhenUnconnected=off
  wires:
  In1/1 -> DummyGain/1
  DummyGain/1 -> Out1/1

== system ASM_Traffic_A11/DomainControl/StartSystem/SignalInterface/ASMSignalInterface/signal_structure ==
  ASMSignalBus : Inport
  BusSelector_1 : BusSelector  OutputSignals=StartButton
  ContentID : Constant  Value=905791938
  DataTypeConversion_1 : DataTypeConversion  OutDataTypeStr=double
  InfoBlock : Subsystem
      mask Display: fprintf('Structural changes of the signal bus require an update \nof the ''ASMSignalCollector'' block. \n\nTo start the update process double click the parent block.\n\n WARNING:\n During update this subsystem will be cleared completely')
  MDLD_DATA_CAPTURE : MDLD_Utils_lib/ModelDeskPlotInterface/DataCapture_Sfcn/MDLD_DATA_CAPTURE  inputPortWidth=6  measurementSignals=[0 0 0 0 0 0]  downsampling=1  samplingPeriod=SIM.StepSize.v  uuid=0  ASMProperties=struct('Name','mdld_data_capture','Version','1.0','Library','mdld_utils_lib')  startTriggerDelay=0  startTriggerLogic=0  startTriggerCount=0  startTriggerConditions=[0,0,0,0,0,0,0,0,0]  stopTriggerDelay=0  stopTriggerLogic=0  stopTriggerCount=0  stopTriggerConditions=[0,0,0,0,0,0,0,0,0]  ContentID_RefStruct=905791938
  SignalFilter : Mux  Inputs=6
  SignalFilterGain : Gain
  StartButton : BusSelector  OutputSignals=Flag_NotPressed_Pedal[0|1],Lock[0|1],Sw_Acc[0|1],Sw_Ignition[0|1],Sw_StarterReq[0|1],State_StartButton[-2|-1|0|1|2|3]
  Terminator : Terminator
  wires:
  ASMSignalBus/1 -> BusSelector_1/1
  BusSelector_1/1 -> StartButton/1  "<StartButton>"
  ContentID/1 -> Terminator/1
  StartButton/1 -> DataTypeConversion_1/1  "<Flag_NotPressed_Pedal[0|1]>"
  DataTypeConversion_1/1 -> SignalFilter/1
  StartButton/2 -> SignalFilter/2  "<Lock[0|1]>"
  StartButton/3 -> SignalFilter/3  "<Sw_Acc[0|1]>"
  StartButton/4 -> SignalFilter/4  "<Sw_Ignition[0|1]>"
  StartButton/5 -> SignalFilter/5  "<Sw_StarterReq[0|1]>"
  StartButton/6 -> SignalFilter/6  "<State_StartButton[-2|-1|0|1|2|3]>"
  SignalFilter/1 -> SignalFilterGain/1
  SignalFilterGain/1 -> MDLD_DATA_CAPTURE/1

== system ASM_Traffic_A11/DomainControl/StartSystem/SignalInterface/ExternalOutports/Select_Outport_Signals ==
  ASMSignalBus : Inport
  Bus Selector : BusSelector  OutputSignals=StartButton.Flag_NotPressed_Pedal[0|1],StartButton.Lock[0|1],StartButton.Sw_Acc[0|1],StartButton.Sw_Ignition[0|1],StartButton.Sw_StarterReq[0|1],StartButton.State_StartButton[-2|-1|0|1|2|3]
  Flag_NotPressed_Pedal[0|1] : Outport  VectorParamsAs1DForOutWhenUnconnected=off
  Lock[0|1] : Outport  Port=2  VectorParamsAs1DForOutWhenUnconnected=off
  Sw_Acc[0|1] : Outport  Port=3  VectorParamsAs1DForOutWhenUnconnected=off
  Sw_Ignition[0|1] : Outport  Port=4  VectorParamsAs1DForOutWhenUnconnected=off
  Sw_StarterReq[0|1] : Outport  Port=5  VectorParamsAs1DForOutWhenUnconnected=off
  State_StartButton[-2|-1|0|1|2|3] : Outport  Port=6  VectorParamsAs1DForOutWhenUnconnected=off
  wires:
  ASMSignalBus/1 -> Bus Selector/1
  Bus Selector/1 -> Flag_NotPressed_Pedal[0|1]/1  "<Flag_NotPressed_Pedal[0|1]>"
  Bus Selector/2 -> Lock[0|1]/1  "<Lock[0|1]>"
  Bus Selector/3 -> Sw_Acc[0|1]/1  "<Sw_Acc[0|1]>"
  Bus Selector/4 -> Sw_Ignition[0|1]/1  "<Sw_Ignition[0|1]>"
  Bus Selector/5 -> Sw_StarterReq[0|1]/1  "<Sw_StarterReq[0|1]>"
  Bus Selector/6 -> State_StartButton[-2|-1|0|1|2|3]/1  "<State_StartButton[-2|-1|0|1|2|3]>"

== system ASM_Traffic_A11/DomainControl/TorqueManager/Control/UserInterface/ASMSignalBus_Control ==
  In : Inport
  Terminator_1 : Terminator
  tag scope: ASMBUS_TorqueManager_Control=global
  wires:
  In/1 -> [ASMBUS_TorqueManager_Control]  "Control"
  [ASMBUS_TorqueManager_Control] -> Terminator_1/1

== system ASM_Traffic_A11/DomainControl/TorqueManager/Control/UserInterface/DISP_Control ==
  In : Inport
  Terminator : Terminator
  wires:
  In/1 -> Terminator/1

== system ASM_Traffic_A11/DomainControl/TorqueManager/Control/UserInterface/PAR_Control ==
  Constant : Constant  Value=0
  Out : Outport  VectorParamsAs1DForOutWhenUnconnected=off
  wires:
  Constant/1 -> Out/1

== system ASM_Traffic_A11/DomainControl/TorqueManager/Interface_In/ModelSignals/Pos_BrakePedal[%]_ ==
  In1 : Inport
  DummyGain : Gain  SaturateOnIntegerOverflow=on  OutDataTypeStr=Inherit: Same as input  ParamDataTypeStr=Inherit: Same as input
  Out1 : Outport  VectorParamsAs1DForOutWhenUnconnected=off
  wires:
  DummyGain/1 -> Out1/1
  In1/1 -> DummyGain/1

== system ASM_Traffic_A11/DomainControl/TorqueManager/Interface_In/ModelSignals/State_Engine[0|1|2|3|4]_ ==
  In1 : Inport
  Gain : Gain  SaturateOnIntegerOverflow=on  OutDataTypeStr=Inherit: Same as input  ParamDataTypeStr=Inherit: Same as input
  Out1 : Outport  VectorParamsAs1DForOutWhenUnconnected=off
  wires:
  In1/1 -> Gain/1
  Gain/1 -> Out1/1

== system ASM_Traffic_A11/DomainControl/TorqueManager/Interface_In/ModelSignals/Sw_Ignition[0|1]_ ==
  In1 : Inport
  DummyGain : Gain  SaturateOnIntegerOverflow=on  OutDataTypeStr=Inherit: Same as input  ParamDataTypeStr=Inherit: Same as input
  Out1 : Outport  VectorParamsAs1DForOutWhenUnconnected=off
  wires:
  In1/1 -> DummyGain/1
  DummyGain/1 -> Out1/1

== system ASM_Traffic_A11/DomainControl/TorqueManager/Interface_In/ModelSignals/Sw_ModelDeskPlottingInterface[0Disabled|1Enabled]_ ==
  In1 : Inport
  Gain : Gain
  Out1 : Outport
  wires:
  Gain/1 -> Out1/1
  In1/1 -> Gain/1

== system ASM_Traffic_A11/DomainControl/TorqueManager/Interface_In/ModelSignals/Sw_ModelPortBlocks[0Disabled|1Enabled]_ ==
  In1 : Inport
  Gain : Gain
  Out1 : Outport
  wires:
  Gain/1 -> Out1/1
  In1/1 -> Gain/1

== system ASM_Traffic_A11/DomainControl/TorqueManager/Interface_In/ModelSignals/Sw_StarterReq[0|1]_ ==
  In1 : Inport
  DummyGain : Gain  SaturateOnIntegerOverflow=on  OutDataTypeStr=Inherit: Same as input  ParamDataTypeStr=Inherit: Same as input
  Out1 : Outport  VectorParamsAs1DForOutWhenUnconnected=off
  wires:
  DummyGain/1 -> Out1/1
  In1/1 -> DummyGain/1

== system ASM_Traffic_A11/DomainControl/TorqueManager/Interface_In/ModelSignals/Sw_Starter[0Off|1On]_ ==
  In1 : Inport
  DummyGain : Gain  SaturateOnIntegerOverflow=on  OutDataTypeStr=Inherit: Same as input  ParamDataTypeStr=Inherit: Same as input
  Out1 : Outport  VectorParamsAs1DForOutWhenUnconnected=off
  wires:
  In1/1 -> DummyGain/1
  DummyGain/1 -> Out1/1

== system ASM_Traffic_A11/DomainControl/TorqueManager/Interface_Out/Control_ModelSignals/ Mode_BSG[-1|0|1|2|3|4|5]_ ==
  In1 : Inport
  Gain : Gain  SaturateOnIntegerOverflow=on  OutDataTypeStr=Inherit: Same as input  ParamDataTypeStr=Inherit: Same as input
  Out1 : Outport  VectorParamsAs1DForOutWhenUnconnected=off
  wires:
  Gain/1 -> Out1/1
  In1/1 -> Gain/1

== system ASM_Traffic_A11/DomainControl/TorqueManager/Interface_Out/Control_ModelSignals/HybridMode_ICE[0Off|1OnIdle|2OnPower|3err]_ ==
  In1 : Inport
  Gain : Gain  SaturateOnIntegerOverflow=on  OutDataTypeStr=Inherit: Same as input  ParamDataTypeStr=Inherit: Same as input
  Out1 : Outport  VectorParamsAs1DForOutWhenUnconnected=off
  wires:
  In1/1 -> Gain/1
  Gain/1 -> Out1/1

== system ASM_Traffic_A11/DomainControl/TorqueManager/Interface_Out/Control_ModelSignals/Ignition_ICE[0Off|1On]_ ==
  In1 : Inport
  Gain : Gain  SaturateOnIntegerOverflow=on  OutDataTypeStr=Inherit: Same as input  ParamDataTypeStr=Inherit: Same as input
  Out1 : Outport  VectorParamsAs1DForOutWhenUnconnected=off
  wires:
  In1/1 -> Gain/1
  Gain/1 -> Out1/1

== system ASM_Traffic_A11/DomainControl/TorqueManager/Interface_Out/Control_ModelSignals/Pos_BrakePedal_Desired[%]_ ==
  In1 : Inport
  Gain : Gain  SaturateOnIntegerOverflow=on  OutDataTypeStr=Inherit: Same as input  ParamDataTypeStr=Inherit: Same as input
  Out1 : Outport  VectorParamsAs1DForOutWhenUnconnected=off
  wires:
  In1/1 -> Gain/1
  Gain/1 -> Out1/1

== system ASM_Traffic_A11/DomainControl/TorqueManager/Interface_Out/Control_ModelSignals/StarterReq_ICE[0Off|1On]_ ==
  In1 : Inport
  Gain : Gain  SaturateOnIntegerOverflow=on  OutDataTypeStr=Inherit: Same as input  ParamDataTypeStr=Inherit: Same as input
  Out1 : Outport  VectorParamsAs1DForOutWhenUnconnected=off
  wires:
  In1/1 -> Gain/1
  Gain/1 -> Out1/1

== system ASM_Traffic_A11/DomainControl/TorqueManager/Interface_Out/Control_ModelSignals/Starter_Drivetrain[0Off|1On]_ ==
  In1 : Inport
  Gain : Gain  SaturateOnIntegerOverflow=on  OutDataTypeStr=Inherit: Same as input  ParamDataTypeStr=Inherit: Same as input
  Out1 : Outport  VectorParamsAs1DForOutWhenUnconnected=off
  wires:
  Gain/1 -> Out1/1
  In1/1 -> Gain/1

== system ASM_Traffic_A11/DomainControl/TorqueManager/Interface_Out/Control_ModelSignals/State_Engine[0|1|2|3|4]_ ==
  In1 : Inport
  Gain : Gain  SaturateOnIntegerOverflow=on  OutDataTypeStr=Inherit: Same as input  ParamDataTypeStr=Inherit: Same as input
  Out1 : Outport  VectorParamsAs1DForOutWhenUnconnected=off
  wires:
  In1/1 -> Gain/1
  Gain/1 -> Out1/1

== system ASM_Traffic_A11/DomainControl/TorqueManager/Interface_Out/Control_ModelSignals/Sw_DriveMode[0Hybrid|1ICE|2EM]_ ==
  In1 : Inport
  Gain : Gain  SaturateOnIntegerOverflow=on  OutDataTypeStr=Inherit: Same as input  ParamDataTypeStr=Inherit: Same as input
  Out1 : Outport  VectorParamsAs1DForOutWhenUnconnected=off
  wires:
  Gain/1 -> Out1/1
  In1/1 -> Gain/1

== system ASM_Traffic_A11/DomainControl/TorqueManager/Interface_Out/Control_ModelSignals/Trq_Request_Brake[Nm]_ ==
  In1 : Inport
  Gain : Gain  SaturateOnIntegerOverflow=on  OutDataTypeStr=Inherit: Same as input  ParamDataTypeStr=Inherit: Same as input
  Out1 : Outport  VectorParamsAs1DForOutWhenUnconnected=off
  wires:
  Gain/1 -> Out1/1
  In1/1 -> Gain/1

== system ASM_Traffic_A11/DomainControl/TorqueManager/Interface_Out/Control_ModelSignals/Trq_Request_EM[Nm]_ ==
  In1 : Inport
  Gain : Gain  SaturateOnIntegerOverflow=on  OutDataTypeStr=Inherit: Same as input  ParamDataTypeStr=Inherit: Same as input
  Out1 : Outport  VectorParamsAs1DForOutWhenUnconnected=off
  wires:
  Gain/1 -> Out1/1
  In1/1 -> Gain/1

== system ASM_Traffic_A11/DomainControl/TorqueManager/Interface_Out/Control_ModelSignals/Trq_Request_ICE[Nm]_ ==
  In1 : Inport
  Gain : Gain  SaturateOnIntegerOverflow=on  OutDataTypeStr=Inherit: Same as input  ParamDataTypeStr=Inherit: Same as input
  Out1 : Outport  VectorParamsAs1DForOutWhenUnconnected=off
  wires:
  In1/1 -> Gain/1
  Gain/1 -> Out1/1

== system ASM_Traffic_A11/DomainControl/TorqueManager/Interface_Out/Control_ModelSignals/Vehicle_Topology[-2|-1|0|2]_ ==
  In1 : Inport
  Gain : Gain  SaturateOnIntegerOverflow=on  OutDataTypeStr=Inherit: Same as input  ParamDataTypeStr=Inherit: Same as input
  Out1 : Outport  VectorParamsAs1DForOutWhenUnconnected=off
  wires:
  Gain/1 -> Out1/1
  In1/1 -> Gain/1

== system ASM_Traffic_A11/DomainControl/TorqueManager/SignalInterface/ASMSignalInterface/signal_structure ==
  ASMSignalBus : Inport
  BusSelector_1 : BusSelector  OutputSignals=ExternalModel
  ContentID : Constant  Value=126986817
  ExternalModel : BusSelector  OutputSignals=Sw_Ignition[0|1],Sw_StarterReq[0|1],Pos_BrakePedal[%],Sw_Starter[0Off|1On],State_Engine[0|1|2|3|4]
  InfoBlock : Subsystem
      mask Display: fprintf('Structural changes of the signal bus require an update \nof the ''ASMSignalCollector'' block. \n\nTo start the update process double click the parent block.\n\n WARNING:\n During update this subsystem will be cleared completely')
  MDLD_DATA_CAPTURE : MDLD_Utils_lib/ModelDeskPlotInterface/DataCapture_Sfcn/MDLD_DATA_CAPTURE  inputPortWidth=5  measurementSignals=[0 0 0 0 0]  downsampling=1  samplingPeriod=SIM.StepSize.v  uuid=0  ASMProperties=struct('Name','mdld_data_capture','Version','1.0','Library','mdld_utils_lib')  startTriggerDelay=0  startTriggerLogic=0  startTriggerCount=0  startTriggerConditions=[0,0,0,0,0,0,0,0,0]  stopTriggerDelay=0  stopTriggerLogic=0  stopTriggerCount=0  stopTriggerConditions=[0,0,0,0,0,0,0,0,0]  ContentID_RefStruct=126986817
  SignalFilter : Mux  Inputs=5
  SignalFilterGain : Gain
  Terminator : Terminator
  wires:
  ASMSignalBus/1 -> BusSelector_1/1
  BusSelector_1/1 -> ExternalModel/1  "<ExternalModel>"
  ContentID/1 -> Terminator/1
  ExternalModel/1 -> SignalFilter/1  "<Sw_Ignition[0|1]>"
  ExternalModel/2 -> SignalFilter/2  "<Sw_StarterReq[0|1]>"
  ExternalModel/3 -> SignalFilter/3  "<Pos_BrakePedal[%]>"
  ExternalModel/4 -> SignalFilter/4  "<Sw_Starter[0Off|1On]>"
  ExternalModel/5 -> SignalFilter/5  "<State_Engine[0|1|2|3|4]>"
  SignalFilter/1 -> SignalFilterGain/1
  SignalFilterGain/1 -> MDLD_DATA_CAPTURE/1

== system ASM_Traffic_A11/DomainControl/TorqueManager/SignalInterface/ExternalOutports/Select_Outport_Signals ==
  ASMSignalBus : Inport
  Bus Selector : BusSelector  OutputSignals=ExternalModel.Pos_BrakePedal[%],ExternalModel.Sw_Ignition[0|1],ExternalModel.State_Engine[0|1|2|3|4],ExternalModel.Sw_StarterReq[0|1],ExternalModel.Sw_Starter[0Off|1On]
  Sw_Ignition[0|1] : Outport  VectorParamsAs1DForOutWhenUnconnected=off
  Pos_BrakePedal[%] : Outport  Port=2  VectorParamsAs1DForOutWhenUnconnected=off
  State_Engine[0|1|2|3|4] : Outport  Port=3  VectorParamsAs1DForOutWhenUnconnected=off
  Sw_StarterReq[0|1] : Outport  Port=4  VectorParamsAs1DForOutWhenUnconnected=off
  Sw_Starter[0Off|1On] : Outport  Port=5  VectorParamsAs1DForOutWhenUnconnected=off
  wires:
  ASMSignalBus/1 -> Bus Selector/1
  Bus Selector/1 -> Pos_BrakePedal[%]/1  "<Pos_BrakePedal[%]>"
  Bus Selector/2 -> Sw_Ignition[0|1]/1  "<Sw_Ignition[0|1]>"
  Bus Selector/3 -> State_Engine[0|1|2|3|4]/1  "<State_Engine[0|1|2|3|4]>"
  Bus Selector/4 -> Sw_StarterReq[0|1]/1  "<Sw_StarterReq[0|1]>"
  Bus Selector/5 -> Sw_Starter[0Off|1On]/1  "<Sw_Starter[0Off|1On]>"

== system ASM_Traffic_A11/Driver/Plant/Driver/LateralController/LatCtrl1_Enable ==
  Interface_In : Inport
  AND : Logic  IconShape=distinctive  AllPortsSameDT=off  OutDataTypeStr=boolean
  Bus Selector5 : BusSelector  OutputSignals=ExternalModel.Sw_LatDriver[1LatCtrl1|2LatCtrl2],ExternalModel.Mode_Steer[1Stim|2Driver|3Fix]
  DriverMode : simulink/Logic and Bit Operations/Compare To Constant  relop===  const=2  OutDataTypeStr=boolean
  LatCtrl1 : simulink/Logic and Bit Operations/Compare To Constant  relop===  const=1  OutDataTypeStr=boolean
  One : Constant  OutDataTypeStr=Inherit: Inherit via back propagation
  Switch : Switch  Criteria=u2 ~= 0  SaturateOnIntegerOverflow=off  InputSameDT=off
  Zero : Constant  Value=0  OutDataTypeStr=Inherit: Inherit via back propagation
  Out1 : Outport  VectorParamsAs1DForOutWhenUnconnected=off
  wires:
  Zero/1 -> Switch/3
  One/1 -> Switch/1
  Switch/1 -> Out1/1
  DriverMode/1 -> AND/2
  Interface_In/1 -> Bus Selector5/1
  LatCtrl1/1 -> AND/1
  Bus Selector5/2 -> DriverMode/1  "<Mode_Steer[1Stim|2Driver|3Fix]>"
  Bus Selector5/1 -> LatCtrl1/1  "<Sw_LatDriver[1LatCtrl1|2LatCtrl2]>"
  AND/1 -> Switch/2

== system ASM_Traffic_A11/Driver/Plant/Driver/LateralController/LatCtrl2_Enable ==
  Interface_In : Inport
  AND : Logic  IconShape=distinctive  AllPortsSameDT=off  OutDataTypeStr=boolean
  Bus Selector5 : BusSelector  OutputSignals=ExternalModel.Sw_LatDriver[1LatCtrl1|2LatCtrl2],ExternalModel.Mode_Steer[1Stim|2Driver|3Fix]
  DriverMode : simulink/Logic and Bit Operations/Compare To Constant  relop===  const=2  OutDataTypeStr=boolean
  LatCtrl2 : simulink/Logic and Bit Operations/Compare To Constant  relop===  const=2  OutDataTypeStr=boolean
  One : Constant  OutDataTypeStr=Inherit: Inherit via back propagation
  Switch : Switch  Criteria=u2 ~= 0  SaturateOnIntegerOverflow=off  InputSameDT=off
  Zero : Constant  Value=0  OutDataTypeStr=Inherit: Inherit via back propagation
  Out1 : Outport  VectorParamsAs1DForOutWhenUnconnected=off
  wires:
  Switch/1 -> Out1/1
  AND/1 -> Switch/2
  One/1 -> Switch/1
  Zero/1 -> Switch/3
  Bus Selector5/1 -> LatCtrl2/1  "<Sw_LatDriver[1LatCtrl1|2LatCtrl2]>"
  Bus Selector5/2 -> DriverMode/1  "<Mode_Steer[1Stim|2Driver|3Fix]>"
  LatCtrl2/1 -> AND/1
  Interface_In/1 -> Bus Selector5/1
  DriverMode/1 -> AND/2

== system ASM_Traffic_A11/Driver/Plant/Driver/LongitudinalController/Default_GearClutch_Mode ==
  note: For automatic transmission, the default value of GearClutch_Mode is set to the Driver Mode
  Mode_Transmission[1|2] : Inport
  GearClutch_Mode[1Stim|2Driver|3OpenClutch|4RefGear] : Inport  Port=2
  Automatic : simulink/Logic and Bit Operations/Compare To Constant  relop===  const=2  OutDataTypeStr=boolean
  GearClutch_Mode[2Driver] : Constant  Value=2
  Multiport Switch : MultiPortSwitch  Inputs=2  SaturateOnIntegerOverflow=off  InputSameDT=off
  Sw_GearClutchMode[1Driver|2Others] : Constant
  Switch : Switch  Criteria=u2 ~= 0  SaturateOnIntegerOverflow=off  InputSameDT=off
  GearClutch_Mode[1Stim|2Driver|3OpenClutch|4RefGear]_ : Outport  OutputWhenDisabled=reset  InitialOutput=0  VectorParamsAs1DForOutWhenUnconnected=off
  wires:
  Mode_Transmission[1|2]/1 -> Automatic/1
  Automatic/1 -> Switch/2
  Switch/1 -> GearClutch_Mode[1Stim|2Driver|3OpenClutch|4RefGear]_/1
  GearClutch_Mode[1Stim|2Driver|3OpenClutch|4RefGear]/1 -> Switch/3, Multiport Switch/3
  GearClutch_Mode[2Driver]/1 -> Multiport Switch/2
  Sw_GearClutchMode[1Driver|2Others]/1 -> Multiport Switch/1
  Multiport Switch/1 -> Switch/1

== system ASM_Traffic_A11/Driver/Plant/Driver/ReferenceVelocity/AdaptationForNegativeSpeed ==
  note: ignore adapt velocity to road for backwards driving
  Mode_AdaptVelocityToRoad[1Off|2On] : Inport
  v_Vehicle_Ref_Maneuver[km|h] : Inport  Port=2
  Compare To Zero : simulink/Logic and Bit Operations/Compare To Zero  relop=<  OutDataTypeStr=boolean
  Off : Constant
  Switch : Switch  Criteria=u2 ~= 0  SaturateOnIntegerOverflow=off  InputSameDT=off
  Out1 : Outport
  wires:
  Off/1 -> Switch/1
  Compare To Zero/1 -> Switch/2
  Mode_AdaptVelocityToRoad[1Off|2On]/1 -> Switch/3
  Switch/1 -> Out1/1
  v_Vehicle_Ref_Maneuver[km|h]/1 -> Compare To Zero/1

== system ASM_Traffic_A11/Driver/Plant/Driver/ReferenceVelocity/Driver_Parameters ==
  a_x_Max[m|s2] : Inport
  a_x_Min[m|s2] : Inport  Port=2
  a_y_Max[m|s2] : Inport  Port=3
  n_GG_Acceleration[-] : Inport  Port=4
  n_GG_Deceleration[-] : Inport  Port=5
  a_z_Max_Deflect[m|s2] : Inport  Port=6
  a_z_Max_Rebound[m|s2] : Inport  Port=7
  t_Preview_vRef[s] : Inport  Port=8
  Dist_OutsideRoad_Margin[m] : Inport  Port=9
  v_x_Ref_OutsideRoad[m|s] : Inport  Port=10
  Sw_Observe_v_Scenery_Lim[1Off|2On] : Inport  Port=11
  Mux3 : Mux  Inputs=11
  Driver_Parameters : Outport  VectorParamsAs1DForOutWhenUnconnected=off
  wires:
  Mux3/1 -> Driver_Parameters/1
  t_Preview_vRef[s]/1 -> Mux3/8
  a_y_Max[m|s2]/1 -> Mux3/3
  n_GG_Deceleration[-]/1 -> Mux3/5
  a_z_Max_Rebound[m|s2]/1 -> Mux3/7
  a_z_Max_Deflect[m|s2]/1 -> Mux3/6
  a_x_Max[m|s2]/1 -> Mux3/1
  Dist_OutsideRoad_Margin[m]/1 -> Mux3/9
  v_x_Ref_OutsideRoad[m|s]/1 -> Mux3/10
  n_GG_Acceleration[-]/1 -> Mux3/4
  a_x_Min[m|s2]/1 -> Mux3/2
  Sw_Observe_v_Scenery_Lim[1Off|2On]/1 -> Mux3/11

== system ASM_Traffic_A11/Driver/Plant/Driver/ReferenceVelocity/Extend_Previews ==
  In : Inport
  Dummy : Constant  Value=0
  Mux : Mux  Inputs=7
  Selector : Selector  InputPortWidth=3  IndexOptions=Index vector (dialog)  Indices=[2]  OutputSizes=1
      settings: AttributesFormatString=|
      | PortWidth = %<InputPortWidth>
      | Indices = %<Indices>
  Vector_s_Preview_Discritization[0.2_0.8] : Gain  Gain=[0.2 0.3 0.4 0.5 0.6 0.7 0.8]
  Out : Outport  VectorParamsAs1DForOutWhenUnconnected=off
  wires:
  Dummy/1 -> Mux/3, Mux/4, Mux/5, Mux/6, Mux/7
  Vector_s_Preview_Discritization[0.2_0.8]/1 -> Mux/1
  Selector/1 -> Vector_s_Preview_Discritization[0.2_0.8]/1
  Mux/1 -> Out/1
  In/1 -> Selector/1, Mux/2

== system ASM_Traffic_A11/Driver/Plant/Driver/ReferenceVelocity/Reduce_Dimension ==
  In : Inport
  Selector : Selector  InputPortWidth=15  IndexOptions=Index vector (dialog)  Indices=[8:10]  OutputSizes=1
      settings: AttributesFormatString=|
      | PortWidth = %<InputPortWidth>
      | Indices = %<Indices>
  Out : Outport  VectorParamsAs1DForOutWhenUnconnected=off
  wires:
  In/1 -> Selector/1
  Selector/1 -> Out/1

== system ASM_Traffic_A11/Driver/Plant/Driver/ReferenceVelocity/Reduce_Dimension1 ==
  In : Inport
  Selector : Selector  InputPortWidth=15  IndexOptions=Index vector (dialog)  Indices=[8:10]  OutputSizes=1
      settings: AttributesFormatString=|
      | PortWidth = %<InputPortWidth>
      | Indices = %<Indices>
  Out : Outport  VectorParamsAs1DForOutWhenUnconnected=off
  wires:
  Selector/1 -> Out/1
  In/1 -> Selector/1

== system ASM_Traffic_A11/Driver/Plant/Driver/ReferenceVelocity/Reduce_Dimension2 ==
  In : Inport
  Selector : Selector  InputPortWidth=15  IndexOptions=Index vector (dialog)  Indices=[8:10]  OutputSizes=1
      settings: AttributesFormatString=|
      | PortWidth = %<InputPortWidth>
      | Indices = %<Indices>
  UnitConversion2 : ASM_Utils_lib/UnitConversion/UnitConversion  Selection=km/h_to_m/s
  Out : Outport  VectorParamsAs1DForOutWhenUnconnected=off
  wires:
  UnitConversion2/1 -> Selector/1
  In/1 -> UnitConversion2/1
  Selector/1 -> Out/1

== system ASM_Traffic_A11/Driver/Plant/Driver/ReferenceVelocity/Reduce_Dimension3 ==
  In : Inport
  Selector : Selector  InputPortWidth=15  IndexOptions=Index vector (dialog)  Indices=[1:10]  OutputSizes=1
      settings: AttributesFormatString=|
      | PortWidth = %<InputPortWidth>
      | Indices = %<Indices>
  Out : Outport  VectorParamsAs1DForOutWhenUnconnected=off
  wires:
  In/1 -> Selector/1
  Selector/1 -> Out/1

== system ASM_Traffic_A11/Driver/Plant/Driver/ReferenceVelocity/Reduce_Dimension4 ==
  In : Inport
  Selector : Selector  InputPortWidth=10  IndexOptions=Index vector (dialog)  Indices=[8:10]  OutputSizes=1
      settings: AttributesFormatString=|
      | PortWidth = %<InputPortWidth>
      | Indices = %<Indices>
  Out : Outport  VectorParamsAs1DForOutWhenUnconnected=off
  wires:
  Selector/1 -> Out/1
  In/1 -> Selector/1

== system ASM_Traffic_A11/Driver/Plant/UserInterface/DISP_Plant/Angle_SteeringWheel[deg] ==
  In1 : Inport
  Out1 : Outport  VectorParamsAs1DForOutWhenUnconnected=off
  wires:
  In1/1 -> Out1/1
